simulink model "s_b2a4x1kf"  (R2018b)
settings: Solver=VariableStepDiscrete  StartTime=0.0  StopTime=100  RelTol=1e-3
undefined symbols (not defined in the file): fft_stages, n_bits_ants, n_bits_xengs
libraries: xbsIndex_r4 x20671, casper_library_misc x69, casper_library_scopes x15, casper_library_delays x8, xbsReplacements_r4 x6, xps_library x4
(part 108 of 212)

== system s_b2a4x1kf/sys0/bf/fbf/duplicate ==
  synci : Inport
  eni : Inport  Port=2
  di : Inport  Port=3
  badi : Inport  Port=4
  timei : Inport  Port=5
  misci : Inport  Port=6
  sim_ld : Inport  Port=7
  sim_type : Inport  Port=8
  Convert1 : xbsIndex_r4/Convert  gui_display_data_type=Fixed-point  arith_type=Unsigned  n_bits=n_bits_in*2  bin_pt=0  float_type=Single  exp_bits=8  fraction_bits=24  quantization=Truncate  overflow=Wrap  en=off  latency=0  pipeline=off  dbl_ovrd=off  block_type=convert
      settings: block_version=11.4
  Counter : xbsIndex_r4/Counter  cnt_type=Free Running  cnt_to=inf  operation=Up  start_count=0  cnt_by_val=1  arith_type="Signed  (2's comp)"  n_bits=stack_bits+ant_bits+freq_bits  bin_pt=0  load_pin=off  rst=on  en=on  explicit_period=on  period=1  use_behavioral_HDL=off  implementation=Fabric  dbl_ovrd=off  block_type=counter
      settings: block_version=11.4
  Delay{,1..3,5} (5 alike) : xbsIndex_r4/Delay  rst=off  infoeditControl=Selection of Reset will increase slice count due to use of real FFs and instead of SRLs  en=off  latency=1  reg_retiming=off  dbl_ovrd=off  block_type=delay
      Delay settings: infoedit=Hardware notes: A delay line is a chain, each link of which is an SRL16 or SRL32 followed by a flip-flop.  block_version=11.4
      Delay1 settings: block_version=11.4
      Delay2 settings: block_version=11.4
      Delay3 settings: block_version=11.4
      Delay5 settings: block_version=11.4
  Mux : xbsIndex_r4/Mux  inputs=2  en=off  latency=1  precision=Full  arith_type=Unsigned  n_bits=16  bin_pt=14  quantization=Truncate  overflow=Wrap  dbl_ovrd=off  block_type=mux
      settings: block_version=11.4
  Register1 : xbsIndex_r4/Register  init=0  rst=off  en=on  dbl_ovrd=off  block_type=register
      settings: block_version=11.4
  Slice : xbsIndex_r4/Slice  nbits=freq_bits  boolean_output=off  mode=Upper Bit Location + Width  bit1=0  base1=MSB of Input  bit0=0  base0=LSB of Input  dbl_ovrd=off  block_type=slice
  beam_replicate : Subsystem  Tag=cmac_delinked  mask(bus_replicate){replication=2^beam_bits, csp_latency=0, misc=off, implementation=core}
      mask prompts: replication "replication factor"; csp_latency "latency"; misc "misc support"; implementation "delay implementation"
      mask help: Output bus formed by replicating input bus a number of times
      mask init:
      | bus_replicate_init(gcb, ...
      |     'replication', replication, ...
      |     'csp_latency', csp_latency, ...
      |     'implementation', implementation, ...
      |     'misc', misc);
      mask TypeOptions implementation: core | behavioral
  pol_replicate : Subsystem  Tag=cmac_delinked  mask(bus_replicate){replication=2^polarisation_bits, csp_latency=0, misc=off, implementation=core}
      mask prompts: replication "replication factor"; csp_latency "latency"; misc "misc support"; implementation "delay implementation"
      mask help: Output bus formed by replicating input bus a number of times
      mask init:
      | bus_replicate_init(gcb, ...
      |     'replication', replication, ...
      |     'csp_latency', csp_latency, ...
      |     'implementation', implementation, ...
      |     'misc', misc);
      mask TypeOptions implementation: core | behavioral
  synco : Outport
  do : Outport  Port=2
  eno : Outport  Port=3
  bado : Outport  Port=4
  timeo : Outport  Port=5
  misco : Outport  Port=6
  wires:
  synci/1 -> Delay/1, Counter/1
  eni/1 -> Counter/2, Delay2/1
  badi/1 -> Delay3/1
  misci/1 -> Delay5/1
  timei/1 -> Delay1/1
  Delay/1 -> synco/1
  Delay3/1 -> bado/1
  Delay5/1 -> misco/1
  Delay1/1 -> timeo/1
  sim_ld/1 -> Register1/2
  sim_type/1 -> Register1/1
  beam_replicate/1(out) -> do/1
  Mux/1 -> beam_replicate/1(in)
  Register1/1 -> Mux/1
  di/1 -> Mux/2
  Counter/1 -> Slice/1
  pol_replicate/1(out) -> Mux/3
  Slice/1 -> Convert1/1
  Convert1/1 -> pol_replicate/1(in)
  Delay2/1 -> eno/1

== system s_b2a4x1kf/sys0/bf/fbf/pipeline1 ==
  d : Inport
  Register0 : xbsIndex_r4/Register  init=0  rst=off  en=off  dbl_ovrd=off  block_type=register
      settings: block_version=11.4
  Register1 : xbsIndex_r4/Register  init=0  rst=off  en=off  dbl_ovrd=off  block_type=register
      settings: block_version=11.4
  q : Outport
  wires:
  Register0/1 -> Register1/1
  d/1 -> Register0/1
  Register1/1 -> q/1

== system s_b2a4x1kf/sys0/bf/fbf/pipeline10 ==
  d : Inport
  Register0 : xbsIndex_r4/Register  init=0  rst=off  en=off  dbl_ovrd=off  block_type=register
      settings: block_version=11.4
  Register1 : xbsIndex_r4/Register  init=0  rst=off  en=off  dbl_ovrd=off  block_type=register
      settings: block_version=11.4
  q : Outport
  wires:
  Register0/1 -> Register1/1
  d/1 -> Register0/1
  Register1/1 -> q/1

== system s_b2a4x1kf/sys0/bf/fbf/pipeline11 ==
  d : Inport
  Register0 : xbsIndex_r4/Register  init=0  rst=off  en=off  dbl_ovrd=off  block_type=register
      settings: block_version=11.4
  Register1 : xbsIndex_r4/Register  init=0  rst=off  en=off  dbl_ovrd=off  block_type=register
      settings: block_version=11.4
  q : Outport
  wires:
  Register0/1 -> Register1/1
  d/1 -> Register0/1
  Register1/1 -> q/1

== system s_b2a4x1kf/sys0/bf/fbf/pipeline12 ==
  d : Inport
  Register0 : xbsIndex_r4/Register  init=0  rst=off  en=off  dbl_ovrd=off  block_type=register
      settings: block_version=11.4
  Register1 : xbsIndex_r4/Register  init=0  rst=off  en=off  dbl_ovrd=off  block_type=register
      settings: block_version=11.4
  q : Outport
  wires:
  Register0/1 -> Register1/1
  d/1 -> Register0/1
  Register1/1 -> q/1

== system s_b2a4x1kf/sys0/bf/fbf/pipeline13 ==
  d : Inport
  Register0 : xbsIndex_r4/Register  init=0  rst=off  en=off  dbl_ovrd=off  block_type=register
      settings: block_version=11.4
  Register1 : xbsIndex_r4/Register  init=0  rst=off  en=off  dbl_ovrd=off  block_type=register
      settings: block_version=11.4
  q : Outport
  wires:
  Register0/1 -> Register1/1
  d/1 -> Register0/1
  Register1/1 -> q/1

== system s_b2a4x1kf/sys0/bf/fbf/pipeline14 ==
  d : Inport
  Register0 : xbsIndex_r4/Register  init=0  rst=off  en=off  dbl_ovrd=off  block_type=register
      settings: block_version=11.4
  Register1 : xbsIndex_r4/Register  init=0  rst=off  en=off  dbl_ovrd=off  block_type=register
      settings: block_version=11.4
  q : Outport
  wires:
  Register0/1 -> Register1/1
  d/1 -> Register0/1
  Register1/1 -> q/1

== system s_b2a4x1kf/sys0/bf/fbf/pipeline15 ==
  d : Inport
  Register0 : xbsIndex_r4/Register  init=0  rst=off  en=off  dbl_ovrd=off  block_type=register
      settings: block_version=11.4
  Register1 : xbsIndex_r4/Register  init=0  rst=off  en=off  dbl_ovrd=off  block_type=register
      settings: block_version=11.4
  q : Outport
  wires:
  Register0/1 -> Register1/1
  d/1 -> Register0/1
  Register1/1 -> q/1

== system s_b2a4x1kf/sys0/bf/fbf/pipeline16 ==
  d : Inport
  Register0 : xbsIndex_r4/Register  init=0  rst=off  en=off  dbl_ovrd=off  block_type=register
      settings: block_version=11.4
  Register1 : xbsIndex_r4/Register  init=0  rst=off  en=off  dbl_ovrd=off  block_type=register
      settings: block_version=11.4
  q : Outport
  wires:
  Register0/1 -> Register1/1
  d/1 -> Register0/1
  Register1/1 -> q/1

== system s_b2a4x1kf/sys0/bf/fbf/pipeline2 ==
  d : Inport
  Register0 : xbsIndex_r4/Register  init=0  rst=off  en=off  dbl_ovrd=off  block_type=register
      settings: block_version=11.4
  Register1 : xbsIndex_r4/Register  init=0  rst=off  en=off  dbl_ovrd=off  block_type=register
      settings: block_version=11.4
  q : Outport
  wires:
  Register0/1 -> Register1/1
  d/1 -> Register0/1
  Register1/1 -> q/1

== system s_b2a4x1kf/sys0/bf/fbf/pipeline3 ==
  d : Inport
  Register0 : xbsIndex_r4/Register  init=0  rst=off  en=off  dbl_ovrd=off  block_type=register
      settings: block_version=11.4
  Register1 : xbsIndex_r4/Register  init=0  rst=off  en=off  dbl_ovrd=off  block_type=register
      settings: block_version=11.4
  q : Outport
  wires:
  Register0/1 -> Register1/1
  d/1 -> Register0/1
  Register1/1 -> q/1

== system s_b2a4x1kf/sys0/bf/fbf/pipeline8 ==
  d : Inport
  Register0 : xbsIndex_r4/Register  init=0  rst=off  en=off  dbl_ovrd=off  block_type=register
      settings: block_version=11.4
  Register1 : xbsIndex_r4/Register  init=0  rst=off  en=off  dbl_ovrd=off  block_type=register
      settings: block_version=11.4
  q : Outport
  wires:
  Register0/1 -> Register1/1
  d/1 -> Register0/1
  Register1/1 -> q/1

== system s_b2a4x1kf/sys0/bf/fbf/pipeline9 ==
  d : Inport
  Register0 : xbsIndex_r4/Register  init=0  rst=off  en=off  dbl_ovrd=off  block_type=register
      settings: block_version=11.4
  Register1 : xbsIndex_r4/Register  init=0  rst=off  en=off  dbl_ovrd=off  block_type=register
      settings: block_version=11.4
  q : Outport
  wires:
  Register0/1 -> Register1/1
  d/1 -> Register0/1
  Register1/1 -> q/1

== system s_b2a4x1kf/sys0/bf/fbf/requantise ==
  synci : Inport
  din : Inport  Port=2
  den : Inport  Port=3
  misci : Inport  Port=4
  vali : Inport  Port=5
  Concat : xbsIndex_r4/Concat  num_inputs=3  dbl_ovrd=off  block_type=concat
  Slice : xbsIndex_r4/Slice  nbits=1  boolean_output=on  mode=Upper Bit Location + Width  bit1=-1  base1=MSB of Input  bit0=0  base0=LSB of Input  dbl_ovrd=off  block_type=slice
  Slice1 : xbsIndex_r4/Slice  nbits=1  boolean_output=off  mode=Two Bit Locations  bit1=-2  base1=MSB of Input  bit0=0  base0=LSB of Input  dbl_ovrd=off  block_type=slice
  Slice2 : xbsIndex_r4/Slice  nbits=1  boolean_output=on  mode=Upper Bit Location + Width  bit1=0  base1=MSB of Input  bit0=0  base0=LSB of Input  dbl_ovrd=off  block_type=slice
  bus_convert : Subsystem  Tag=cmac_delinked  mask(bus_convert){n_bits_in=repmat(n_bits_coeff+n_bits_in+1, 1, 2^stream_bits), bin_pt_in=bin_pt_coeff+bin_pt_in, cmplx=on, n_bits_out=n_bits_out, bin_pt_out=bin_pt_out, quantization=quantization, overflow=overflow, csp_latency=conv_latency, of=off, misc=on}
      mask prompts: n_bits_in "input bit widths"; bin_pt_in "input binary points"; cmplx "input complex"; n_bits_out "output bit widths"; bin_pt_out "output binary points"; quantization "quantization strategy (Truncate=0, Round  (unbiased: +/- Inf)=1, Round (unbiased: Even Values)=2)"; overflow "overflow strategy (Wrap=0, Saturate=1, Flag as error=2)"; csp_latency "latency"; of "overflow indication"; misc "misc support"
      mask help: Convert components of busses
      mask init: same as s_b2a4x1kf/sys0/31->32
  bus_mult : Subsystem  mask(bus_mult){n_bits_a=repmat(n_bits_in, 1, 2^stream_bits), bin_pt_a=bin_pt_in, type_a=type_in, cmplx_a=on, n_bits_b=repmat(n_bits_coeff, 1, 2^stream_bits), bin_pt_b=bin_pt_coeff, type_b=type_coeff, cmplx_b=off, n_bits_out=n_bits_coeff+n_bits_in+1, bin_pt_out=bin_pt_coeff+bin_pt_in, type_out=type_out, quantization=0, overflow=0, mult_latency=mult_latency, add_latency=2, conv_latency=0, max_fanout=2, fan_latency=1, multiplier_implementation=embedded multiplier core, misc=on}
      mask prompts: n_bits_a "a input bit widths"; bin_pt_a "a input binary points"; type_a "a input type (Unsigned=0, Signed=1)"; cmplx_a "a input complex"; n_bits_b "b input bit widths"; bin_pt_b "b input binary points"; type_b "b input type (Unsigned=0, Signed=1)"; cmplx_b "b input complex"; n_bits_out "output bit widths"; bin_pt_out "output binary points"; type_out "output type (Unsigned=0, Signed=1)"; quantization "quantization strategy (Truncate=0, Round  (unbiased: +/- Inf)=1)"; overflow "overflow strategy (Wrap=0, Saturate=1, Flag as error=2)"; mult_latency "multiplier latency"; add_latency "adder latency"; conv_latency "convert latency"; max_fanout "limit fanout to ?"; fan_latency "fanout register latency"; multiplier_implementation "multiplier implementation"; misc "misc support"
      mask help: Multiply components of two busses
      mask init: same as s_b2a4x1kf/sys0/bf/fbf/apply_beam_weights/bus_mult
      mask TypeOptions multiplier_implementation: behavioral HDL | standard core | embedded multiplier core
  synco : Outport
  dout : Outport  Port=2
  eno : Outport  Port=3
  misco : Outport  Port=4
  wires:
  bus_convert/1(dout) -> dout/1
  vali/1 -> bus_mult/2(b)
  Slice2/1 -> synco/1
  misci/1 -> Concat/3
  bus_convert/2(misco) -> Slice1/1, Slice2/1, Slice/1
  Slice1/1 -> misco/1
  Slice/1 -> eno/1
  synci/1 -> Concat/1
  den/1 -> Concat/2
  din/1 -> bus_mult/1(a)
  bus_mult/1(a*b) -> bus_convert/1(din)
  Concat/1 -> bus_mult/3(misci)
  bus_mult/2(misco) -> bus_convert/2(misci)

== system s_b2a4x1kf/sys0/bf/fbf/sync_gen ==
  en : Inport
  di : Inport  Port=2
  badi : Inport  Port=3
  timei : Inport  Port=4
  misci : Inport  Port=5
  Delay{,1..10} (11 alike) : xbsIndex_r4/Delay  rst=off  infoeditControl=Selection of Reset will increase slice count due to use of real FFs and instead of SRLs  en=off  latency=1  reg_retiming=on  dbl_ovrd=off  block_type=delay
  different_time : xbsIndex_r4/Relational  mode=a!=b  op_type=Bool  en=off  latency=0  dbl_ovrd=off  block_type=relational
  pre_time : xbsIndex_r4/Register  init=0  rst=off  en=off  dbl_ovrd=off  block_type=register
  synco : Outport
  do : Outport  Port=2
  dvalid : Outport  Port=3
  bado : Outport  Port=4
  timeo : Outport  Port=5
  misco : Outport  Port=6
  wires:
  Delay9/1 -> misco/1
  Delay7/1 -> bado/1
  Delay8/1 -> do/1
  Delay3/1 -> Delay9/1
  Delay2/1 -> Delay7/1
  Delay1/1 -> Delay8/1
  Delay4/1 -> dvalid/1
  Delay6/1 -> timeo/1
  Delay5/1 -> Delay6/1
  different_time/1 -> Delay10/1
  Delay/1 -> Delay4/1
  badi/1 -> Delay2/1
  misci/1 -> Delay3/1
  di/1 -> Delay1/1
  en/1 -> Delay/1
  pre_time/1 -> different_time/2
  timei/1 -> Delay5/1, pre_time/1, different_time/1
  Delay10/1 -> synco/1

== system s_b2a4x1kf/sys0/bf_pack_out0/Subsystem3/edge_detect ==
  in : Inport
  Delay : xbsIndex_r4/Delay  rst=off  infoeditControl=Selection of Reset will increase slice count due to use of real FFs and instead of SRLs  en=off  latency=1  reg_retiming=off  dbl_ovrd=off  block_type=delay
      settings: xl_area=[0, 0, 0, 0, 0, 0, 0]
  Inverter : xbsIndex_r4/Inverter  en=off  latency=0  dbl_ovrd=off  block_type=inv
      settings: xl_area=[0, 0, 0, 0, 0, 0, 0]
  edge_op : xbsIndex_r4/Logical  logical_function=NOR  inputs=2  en=off  latency=0  precision=Full  arith_type=Unsigned  n_bits=8  bin_pt=2  align_bp=on  dbl_ovrd=off  block_type=logical
      settings: xl_area=[0, 0, 0, 0, 0, 0, 0]
  out : Outport
  wires:
  Inverter/1 -> edge_op/1
  edge_op/1 -> out/1
  in/1 -> Inverter/1, Delay/1
  Delay/1 -> edge_op/2

== system s_b2a4x1kf/sys0/bf_pack_out0/Subsystem3/edge_detect1 ==
  in : Inport
  Delay : xbsIndex_r4/Delay  rst=off  infoeditControl=Selection of Reset will increase slice count due to use of real FFs and instead of SRLs  en=off  latency=1  reg_retiming=off  dbl_ovrd=off  block_type=delay
      settings: xl_area=[0, 0, 0, 0, 0, 0, 0]
  Inverter : xbsIndex_r4/Inverter  en=off  latency=0  dbl_ovrd=off  block_type=inv
      settings: xl_area=[0, 0, 0, 0, 0, 0, 0]
  edge_op : xbsIndex_r4/Logical  logical_function=NOR  inputs=2  en=off  latency=0  precision=Full  arith_type=Unsigned  n_bits=8  bin_pt=2  align_bp=on  dbl_ovrd=off  block_type=logical
      settings: xl_area=[0, 0, 0, 0, 0, 0, 0]
  out : Outport
  wires:
  Inverter/1 -> edge_op/1
  edge_op/1 -> out/1
  in/1 -> Inverter/1, Delay/1
  Delay/1 -> edge_op/2

== system s_b2a4x1kf/sys0/bf_pack_out0/Subsystem3/pipeline1 ==
  d : Inport
  Register0 : xbsIndex_r4/Register  init=0  rst=off  en=off  dbl_ovrd=off  block_type=register
      settings: block_version=11.4
  Register1 : xbsIndex_r4/Register  init=0  rst=off  en=off  dbl_ovrd=off  block_type=register
      settings: block_version=11.4
  q : Outport
  wires:
  Register0/1 -> Register1/1
  d/1 -> Register0/1
  Register1/1 -> q/1

== system s_b2a4x1kf/sys0/bf_pack_out0/Subsystem3/pipeline2 ==
  d : Inport
  Register0 : xbsIndex_r4/Register  init=0  rst=off  en=off  dbl_ovrd=off  block_type=register
      settings: block_version=11.4
  Register1 : xbsIndex_r4/Register  init=0  rst=off  en=off  dbl_ovrd=off  block_type=register
      settings: block_version=11.4
  q : Outport
  wires:
  Register0/1 -> Register1/1
  d/1 -> Register0/1
  Register1/1 -> q/1

== system s_b2a4x1kf/sys0/bf_pack_out0/Subsystem3/pipeline53 ==
  d : Inport
  Register0 : xbsIndex_r4/Register  init=0  rst=off  en=off  dbl_ovrd=off  block_type=register
      settings: block_version=11.4
  Register1 : xbsIndex_r4/Register  init=0  rst=off  en=off  dbl_ovrd=off  block_type=register
      settings: block_version=11.4
  q : Outport
  wires:
  Register0/1 -> Register1/1
  d/1 -> Register0/1
  Register1/1 -> q/1

== system s_b2a4x1kf/sys0/bf_pack_out0/Subsystem3/pipeline54 ==
  d : Inport
  Register0 : xbsIndex_r4/Register  init=0  rst=off  en=off  dbl_ovrd=off  block_type=register
      settings: block_version=11.4
  Register1 : xbsIndex_r4/Register  init=0  rst=off  en=off  dbl_ovrd=off  block_type=register
      settings: block_version=11.4
  q : Outport
  wires:
  Register0/1 -> Register1/1
  d/1 -> Register0/1
  Register1/1 -> q/1

== system s_b2a4x1kf/sys0/bf_pack_out0/Subsystem3/pipeline55 ==
  d : Inport
  Register0 : xbsIndex_r4/Register  init=0  rst=off  en=off  dbl_ovrd=off  block_type=register
      settings: block_version=11.4
  Register1 : xbsIndex_r4/Register  init=0  rst=off  en=off  dbl_ovrd=off  block_type=register
      settings: block_version=11.4
  q : Outport
  wires:
  Register0/1 -> Register1/1
  d/1 -> Register0/1
  Register1/1 -> q/1

== system s_b2a4x1kf/sys0/bf_pack_out0/Subsystem3/pipeline7 ==
  d : Inport
  Register0 : xbsIndex_r4/Register  init=0  rst=off  en=off  dbl_ovrd=off  block_type=register
      settings: block_version=11.4
  Register1 : xbsIndex_r4/Register  init=0  rst=off  en=off  dbl_ovrd=off  block_type=register
      settings: block_version=11.4
  q : Outport
  wires:
  Register0/1 -> Register1/1
  d/1 -> Register0/1
  Register1/1 -> q/1

== system s_b2a4x1kf/sys0/bf_pack_out0/data_fifo/bus_replicate ==
  in : Inport
  bussify : Subsystem  mask(bus_create){inputNum=16}
      mask prompts: inputNum "Number of inputs:"
      mask init:
      | bus_create_init(gcb,...
      |     'inputNum', inputNum);
  out : Outport
  wires:
  in/1 -> bussify/1(in1), bussify/2(in2), bussify/3(in3), bussify/4(in4), bussify/5(in5), bussify/6(in6), bussify/7(in7), bussify/8(in8), bussify/9(in9), bussify/10(in10), bussify/11(in11), bussify/12(in12), bussify/13(in13), bussify/14(in14), bussify/15(in15), bussify/16(in16)
  bussify/1(bus_out) -> out/1

== system s_b2a4x1kf/sys0/bf_pack_out0/data_fifo/edge_detect ==
  in : Inport
  Delay : xbsIndex_r4/Delay  rst=off  infoeditControl=Selection of Reset will increase slice count due to use of real FFs and instead of SRLs  en=off  latency=1  reg_retiming=on  dbl_ovrd=off  block_type=delay
      settings: xl_area=[0, 0, 0, 0, 0, 0, 0]
  Inverter : xbsIndex_r4/Inverter  en=off  latency=0  dbl_ovrd=off  block_type=inv
      settings: xl_area=[0, 0, 0, 0, 0, 0, 0]
  edge_op : xbsIndex_r4/Logical  logical_function=AND  inputs=2  en=off  latency=0  precision=Full  arith_type=Unsigned  n_bits=8  bin_pt=2  align_bp=on  dbl_ovrd=off  block_type=logical
      settings: xl_area=[0, 0, 0, 0, 0, 0, 0]
  out : Outport
  wires:
  Inverter/1 -> edge_op/1
  edge_op/1 -> out/1
  in/1 -> Inverter/1, Delay/1
  Delay/1 -> edge_op/2

== system s_b2a4x1kf/sys0/bf_pack_out0/data_fifo/edge_detect1 ==
  in : Inport
  Delay : xbsIndex_r4/Delay  rst=off  infoeditControl=Selection of Reset will increase slice count due to use of real FFs and instead of SRLs  en=off  latency=1  reg_retiming=on  dbl_ovrd=off  block_type=delay
      settings: xl_area=[0, 0, 0, 0, 0, 0, 0]
  Inverter : xbsIndex_r4/Inverter  en=off  latency=0  dbl_ovrd=off  block_type=inv
      settings: xl_area=[0, 0, 0, 0, 0, 0, 0]
  edge_op : xbsIndex_r4/Logical  logical_function=AND  inputs=2  en=off  latency=0  precision=Full  arith_type=Unsigned  n_bits=8  bin_pt=2  align_bp=on  dbl_ovrd=off  block_type=logical
      settings: xl_area=[0, 0, 0, 0, 0, 0, 0]
  out : Outport
  wires:
  Delay/1 -> edge_op/2
  in/1 -> Delay/1, Inverter/1
  edge_op/1 -> out/1
  Inverter/1 -> edge_op/1

== system s_b2a4x1kf/sys0/bf_pack_out0/data_fifo/munge ==
  din : Inport
  join : Subsystem  mask(bus_create){inputNum=16}
      mask prompts: inputNum "Number of inputs:"
      mask init:
      | bus_create_init(gcb,...
      |     'inputNum', inputNum);
  reinterpret : xbsIndex_r4/Reinterpret  force_arith_type=on  arith_type=Unsigned  force_bin_pt=on  bin_pt=0  block_type=reinterpret
      settings: infoedit="Changes signal type without altering the binary representation.   You can changed the signal between signed and unsigned, and relocate the binary point.<br><br>Hardware notes: In hardware this block costs nothing.<br><br>Example:  Suppose the input is 6 bits wide, signed, with 2 fractional bits, and the output is forced to unsigned with 0 fractional bits.  Then an input of -2.0 (1110.00 in binary 2's complement) becomes an output of 56 (111000 in binary)."
  reinterpret_out : xbsIndex_r4/Reinterpret  force_arith_type=on  arith_type=Unsigned  force_bin_pt=on  bin_pt=0  block_type=reinterpret
  split : Subsystem  mask(bus_expand){mode=divisions of arbitrary size, outputNum=1, outputWidth=[16 16 16 16 16 16 16 16 16 16 16 16 16 16 16 16], outputBinaryPt=[0 0 0 0 0 0 0 0 0 0 0 0 0 0 0 0], outputArithmeticType=[0 0 0 0 0 0 0 0 0 0 0 0 0 0 0 0], show_format=off, outputToWorkspace=off, variablePrefix=out, outputToModelAsWell=on}
      mask prompts: outputNum "Number of outputs:"; outputWidth "Output width [msb ... lsb]:"; outputBinaryPt "Output binary point position [msb ... lsb]:"; outputArithmeticType "Output arithmetic type (ufix=0, fix=1, bool=2) [msb ... lsb]:"; show_format "Print format string?"; outputToWorkspace "Output to workspace?"; variablePrefix "Variable name prefix:"; outputToModelAsWell "Output to model as well?"
      mask help:
      | Expands a 'bus' made using a bus_create or Xilinx
      | concat block.
      | The input will be divided into the specified number
      | of outputs with the specified arithmetic types.
      | Divisions are made from most significant bit.
      mask init: same as s_b2a4x1kf/bus_expand
      settings: AttributesFormatString=16 outputs
      mask TypeOptions mode: divisions of equal size | divisions of arbitrary size
      mask Callback mode: bus_expand_callback();
      mask Callback outputWidth: bus_expand_callback();
      mask Callback outputToWorkspace: bus_expand_callback();
  dout : Outport
  wires:
  reinterpret_out/1 -> dout/1
  din/1 -> reinterpret/1
  reinterpret/1 -> split/1(bus_in)
  join/1(bus_out) -> reinterpret_out/1
  split/16(lsb_out1) -> join/1(in1)
  split/15(out2) -> join/2(in2)
  split/14(out3) -> join/3(in3)
  split/13(out4) -> join/4(in4)
  split/12(out5) -> join/5(in5)
  split/11(out6) -> join/6(in6)
  split/10(out7) -> join/7(in7)
  split/9(out8) -> join/8(in8)
  split/8(out9) -> join/9(in9)
  split/7(out10) -> join/10(in10)
  split/6(out11) -> join/11(in11)
  split/5(out12) -> join/12(in12)
  split/4(out13) -> join/13(in13)
  split/3(out14) -> join/14(in14)
  split/2(out15) -> join/15(in15)
  split/1(msb_out16) -> join/16(in16)

== system s_b2a4x1kf/sys0/bf_pack_out0/pack/edge_detect1 ==
  in : Inport
  Delay : xbsIndex_r4/Delay  rst=off  infoeditControl=Selection of Reset will increase slice count due to use of real FFs and instead of SRLs  en=off  latency=1  reg_retiming=on  dbl_ovrd=off  block_type=delay
      settings: xl_area=[0, 0, 0, 0, 0, 0, 0]
  Inverter : xbsIndex_r4/Inverter  en=off  latency=0  dbl_ovrd=off  block_type=inv
      settings: xl_area=[0, 0, 0, 0, 0, 0, 0]
  edge_op : xbsIndex_r4/Logical  logical_function=AND  inputs=2  en=off  latency=0  precision=Full  arith_type=Unsigned  n_bits=8  bin_pt=2  align_bp=on  dbl_ovrd=off  block_type=logical
      settings: xl_area=[0, 0, 0, 0, 0, 0, 0]
  out : Outport
  wires:
  Delay/1 -> edge_op/2
  in/1 -> Delay/1, Inverter/1
  edge_op/1 -> out/1
  Inverter/1 -> edge_op/1

== system s_b2a4x1kf/sys0/bf_pack_out0/pack/edge_detect3 ==
  in : Inport
  Delay : xbsIndex_r4/Delay  rst=off  infoeditControl=Selection of Reset will increase slice count due to use of real FFs and instead of SRLs  en=off  latency=1  reg_retiming=on  dbl_ovrd=off  block_type=delay
      settings: xl_area=[0, 0, 0, 0, 0, 0, 0]
  Inverter : xbsIndex_r4/Inverter  en=off  latency=0  dbl_ovrd=off  block_type=inv
      settings: xl_area=[0, 0, 0, 0, 0, 0, 0]
  edge_op : xbsIndex_r4/Logical  logical_function=NOR  inputs=2  en=off  latency=0  precision=Full  arith_type=Unsigned  n_bits=8  bin_pt=2  align_bp=on  dbl_ovrd=off  block_type=logical
      settings: xl_area=[0, 0, 0, 0, 0, 0, 0]
  out : Outport
  wires:
  Delay/1 -> edge_op/2
  in/1 -> Delay/1, Inverter/1
  edge_op/1 -> out/1
  Inverter/1 -> edge_op/1

== system s_b2a4x1kf/sys0/bf_pack_out1/Subsystem3/edge_detect ==
  in : Inport
  Delay : xbsIndex_r4/Delay  rst=off  infoeditControl=Selection of Reset will increase slice count due to use of real FFs and instead of SRLs  en=off  latency=1  reg_retiming=off  dbl_ovrd=off  block_type=delay
      settings: xl_area=[0, 0, 0, 0, 0, 0, 0]
  Inverter : xbsIndex_r4/Inverter  en=off  latency=0  dbl_ovrd=off  block_type=inv
      settings: xl_area=[0, 0, 0, 0, 0, 0, 0]
  edge_op : xbsIndex_r4/Logical  logical_function=NOR  inputs=2  en=off  latency=0  precision=Full  arith_type=Unsigned  n_bits=8  bin_pt=2  align_bp=on  dbl_ovrd=off  block_type=logical
      settings: xl_area=[0, 0, 0, 0, 0, 0, 0]
  out : Outport
  wires:
  Inverter/1 -> edge_op/1
  edge_op/1 -> out/1
  in/1 -> Inverter/1, Delay/1
  Delay/1 -> edge_op/2

== system s_b2a4x1kf/sys0/bf_pack_out1/Subsystem3/edge_detect1 ==
  in : Inport
  Delay : xbsIndex_r4/Delay  rst=off  infoeditControl=Selection of Reset will increase slice count due to use of real FFs and instead of SRLs  en=off  latency=1  reg_retiming=off  dbl_ovrd=off  block_type=delay
      settings: xl_area=[0, 0, 0, 0, 0, 0, 0]
  Inverter : xbsIndex_r4/Inverter  en=off  latency=0  dbl_ovrd=off  block_type=inv
      settings: xl_area=[0, 0, 0, 0, 0, 0, 0]
  edge_op : xbsIndex_r4/Logical  logical_function=NOR  inputs=2  en=off  latency=0  precision=Full  arith_type=Unsigned  n_bits=8  bin_pt=2  align_bp=on  dbl_ovrd=off  block_type=logical
      settings: xl_area=[0, 0, 0, 0, 0, 0, 0]
  out : Outport
  wires:
  Inverter/1 -> edge_op/1
  edge_op/1 -> out/1
  in/1 -> Inverter/1, Delay/1
  Delay/1 -> edge_op/2

== system s_b2a4x1kf/sys0/bf_pack_out1/Subsystem3/pipeline1 ==
  d : Inport
  Register0 : xbsIndex_r4/Register  init=0  rst=off  en=off  dbl_ovrd=off  block_type=register
      settings: block_version=11.4
  Register1 : xbsIndex_r4/Register  init=0  rst=off  en=off  dbl_ovrd=off  block_type=register
      settings: block_version=11.4
  q : Outport
  wires:
  Register0/1 -> Register1/1
  d/1 -> Register0/1
  Register1/1 -> q/1

== system s_b2a4x1kf/sys0/bf_pack_out1/Subsystem3/pipeline2 ==
  d : Inport
  Register0 : xbsIndex_r4/Register  init=0  rst=off  en=off  dbl_ovrd=off  block_type=register
      settings: block_version=11.4
  Register1 : xbsIndex_r4/Register  init=0  rst=off  en=off  dbl_ovrd=off  block_type=register
      settings: block_version=11.4
  q : Outport
  wires:
  Register0/1 -> Register1/1
  d/1 -> Register0/1
  Register1/1 -> q/1

== system s_b2a4x1kf/sys0/bf_pack_out1/Subsystem3/pipeline53 ==
  d : Inport
  Register0 : xbsIndex_r4/Register  init=0  rst=off  en=off  dbl_ovrd=off  block_type=register
      settings: block_version=11.4
  Register1 : xbsIndex_r4/Register  init=0  rst=off  en=off  dbl_ovrd=off  block_type=register
      settings: block_version=11.4
  q : Outport
  wires:
  Register0/1 -> Register1/1
  d/1 -> Register0/1
  Register1/1 -> q/1

== system s_b2a4x1kf/sys0/bf_pack_out1/Subsystem3/pipeline54 ==
  d : Inport
  Register0 : xbsIndex_r4/Register  init=0  rst=off  en=off  dbl_ovrd=off  block_type=register
      settings: block_version=11.4
  Register1 : xbsIndex_r4/Register  init=0  rst=off  en=off  dbl_ovrd=off  block_type=register
      settings: block_version=11.4
  q : Outport
  wires:
  Register0/1 -> Register1/1
  d/1 -> Register0/1
  Register1/1 -> q/1

== system s_b2a4x1kf/sys0/bf_pack_out1/Subsystem3/pipeline55 ==
  d : Inport
  Register0 : xbsIndex_r4/Register  init=0  rst=off  en=off  dbl_ovrd=off  block_type=register
      settings: block_version=11.4
  Register1 : xbsIndex_r4/Register  init=0  rst=off  en=off  dbl_ovrd=off  block_type=register
      settings: block_version=11.4
  q : Outport
  wires:
  Register0/1 -> Register1/1
  d/1 -> Register0/1
  Register1/1 -> q/1

== system s_b2a4x1kf/sys0/bf_pack_out1/Subsystem3/pipeline7 ==
  d : Inport
  Register0 : xbsIndex_r4/Register  init=0  rst=off  en=off  dbl_ovrd=off  block_type=register
      settings: block_version=11.4
  Register1 : xbsIndex_r4/Register  init=0  rst=off  en=off  dbl_ovrd=off  block_type=register
      settings: block_version=11.4
  q : Outport
  wires:
  Register0/1 -> Register1/1
  d/1 -> Register0/1
  Register1/1 -> q/1

== system s_b2a4x1kf/sys0/bf_pack_out1/data_fifo/bus_replicate ==
  in : Inport
  bussify : Subsystem  mask(bus_create){inputNum=16}
      mask prompts: inputNum "Number of inputs:"
      mask init:
      | bus_create_init(gcb,...
      |     'inputNum', inputNum);
  out : Outport
  wires:
  in/1 -> bussify/1(in1), bussify/2(in2), bussify/3(in3), bussify/4(in4), bussify/5(in5), bussify/6(in6), bussify/7(in7), bussify/8(in8), bussify/9(in9), bussify/10(in10), bussify/11(in11), bussify/12(in12), bussify/13(in13), bussify/14(in14), bussify/15(in15), bussify/16(in16)
  bussify/1(bus_out) -> out/1

== system s_b2a4x1kf/sys0/bf_pack_out1/data_fifo/edge_detect ==
  in : Inport
  Delay : xbsIndex_r4/Delay  rst=off  infoeditControl=Selection of Reset will increase slice count due to use of real FFs and instead of SRLs  en=off  latency=1  reg_retiming=on  dbl_ovrd=off  block_type=delay
      settings: xl_area=[0, 0, 0, 0, 0, 0, 0]
  Inverter : xbsIndex_r4/Inverter  en=off  latency=0  dbl_ovrd=off  block_type=inv
      settings: xl_area=[0, 0, 0, 0, 0, 0, 0]
  edge_op : xbsIndex_r4/Logical  logical_function=AND  inputs=2  en=off  latency=0  precision=Full  arith_type=Unsigned  n_bits=8  bin_pt=2  align_bp=on  dbl_ovrd=off  block_type=logical
      settings: xl_area=[0, 0, 0, 0, 0, 0, 0]
  out : Outport
  wires:
  Delay/1 -> edge_op/2
  in/1 -> Delay/1, Inverter/1
  edge_op/1 -> out/1
  Inverter/1 -> edge_op/1

== system s_b2a4x1kf/sys0/bf_pack_out1/data_fifo/edge_detect1 ==
  in : Inport
  Delay : xbsIndex_r4/Delay  rst=off  infoeditControl=Selection of Reset will increase slice count due to use of real FFs and instead of SRLs  en=off  latency=1  reg_retiming=on  dbl_ovrd=off  block_type=delay
      settings: xl_area=[0, 0, 0, 0, 0, 0, 0]
  Inverter : xbsIndex_r4/Inverter  en=off  latency=0  dbl_ovrd=off  block_type=inv
      settings: xl_area=[0, 0, 0, 0, 0, 0, 0]
  edge_op : xbsIndex_r4/Logical  logical_function=AND  inputs=2  en=off  latency=0  precision=Full  arith_type=Unsigned  n_bits=8  bin_pt=2  align_bp=on  dbl_ovrd=off  block_type=logical
      settings: xl_area=[0, 0, 0, 0, 0, 0, 0]
  out : Outport
  wires:
  Inverter/1 -> edge_op/1
  edge_op/1 -> out/1
  in/1 -> Inverter/1, Delay/1
  Delay/1 -> edge_op/2

== system s_b2a4x1kf/sys0/bf_pack_out1/data_fifo/munge ==
  din : Inport
  join : Subsystem  mask(bus_create){inputNum=16}
      mask prompts: inputNum "Number of inputs:"
      mask init:
      | bus_create_init(gcb,...
      |     'inputNum', inputNum);
  reinterpret : xbsIndex_r4/Reinterpret  force_arith_type=on  arith_type=Unsigned  force_bin_pt=on  bin_pt=0  block_type=reinterpret
      settings: infoedit="Changes signal type without altering the binary representation.   You can changed the signal between signed and unsigned, and relocate the binary point.<br><br>Hardware notes: In hardware this block costs nothing.<br><br>Example:  Suppose the input is 6 bits wide, signed, with 2 fractional bits, and the output is forced to unsigned with 0 fractional bits.  Then an input of -2.0 (1110.00 in binary 2's complement) becomes an output of 56 (111000 in binary)."
  reinterpret_out : xbsIndex_r4/Reinterpret  force_arith_type=on  arith_type=Unsigned  force_bin_pt=on  bin_pt=0  block_type=reinterpret
  split : Subsystem  mask(bus_expand){mode=divisions of arbitrary size, outputNum=1, outputWidth=[16 16 16 16 16 16 16 16 16 16 16 16 16 16 16 16], outputBinaryPt=[0 0 0 0 0 0 0 0 0 0 0 0 0 0 0 0], outputArithmeticType=[0 0 0 0 0 0 0 0 0 0 0 0 0 0 0 0], show_format=off, outputToWorkspace=off, variablePrefix=out, outputToModelAsWell=on}
      mask prompts: outputNum "Number of outputs:"; outputWidth "Output width [msb ... lsb]:"; outputBinaryPt "Output binary point position [msb ... lsb]:"; outputArithmeticType "Output arithmetic type (ufix=0, fix=1, bool=2) [msb ... lsb]:"; show_format "Print format string?"; outputToWorkspace "Output to workspace?"; variablePrefix "Variable name prefix:"; outputToModelAsWell "Output to model as well?"
      mask help:
      | Expands a 'bus' made using a bus_create or Xilinx
      | concat block.
      | The input will be divided into the specified number
      | of outputs with the specified arithmetic types.
      | Divisions are made from most significant bit.
      mask init: same as s_b2a4x1kf/bus_expand
      settings: AttributesFormatString=16 outputs
      mask TypeOptions mode: divisions of equal size | divisions of arbitrary size
      mask Callback mode: bus_expand_callback();
      mask Callback outputWidth: bus_expand_callback();
      mask Callback outputToWorkspace: bus_expand_callback();
  dout : Outport
  wires:
  split/1(msb_out16) -> join/16(in16)
  split/2(out15) -> join/15(in15)
  split/3(out14) -> join/14(in14)
  split/4(out13) -> join/13(in13)
  split/5(out12) -> join/12(in12)
  split/6(out11) -> join/11(in11)
  split/7(out10) -> join/10(in10)
  split/8(out9) -> join/9(in9)
  split/9(out8) -> join/8(in8)
  split/10(out7) -> join/7(in7)
  split/11(out6) -> join/6(in6)
  split/12(out5) -> join/5(in5)
  split/13(out4) -> join/4(in4)
  split/14(out3) -> join/3(in3)
  split/15(out2) -> join/2(in2)
  split/16(lsb_out1) -> join/1(in1)
  join/1(bus_out) -> reinterpret_out/1
  reinterpret/1 -> split/1(bus_in)
  din/1 -> reinterpret/1
  reinterpret_out/1 -> dout/1

== system s_b2a4x1kf/sys0/bf_pack_out1/pack/edge_detect1 ==
  in : Inport
  Delay : xbsIndex_r4/Delay  rst=off  infoeditControl=Selection of Reset will increase slice count due to use of real FFs and instead of SRLs  en=off  latency=1  reg_retiming=on  dbl_ovrd=off  block_type=delay
      settings: xl_area=[0, 0, 0, 0, 0, 0, 0]
  Inverter : xbsIndex_r4/Inverter  en=off  latency=0  dbl_ovrd=off  block_type=inv
      settings: xl_area=[0, 0, 0, 0, 0, 0, 0]
  edge_op : xbsIndex_r4/Logical  logical_function=AND  inputs=2  en=off  latency=0  precision=Full  arith_type=Unsigned  n_bits=8  bin_pt=2  align_bp=on  dbl_ovrd=off  block_type=logical
      settings: xl_area=[0, 0, 0, 0, 0, 0, 0]
  out : Outport
  wires:
  Inverter/1 -> edge_op/1
  edge_op/1 -> out/1
  in/1 -> Inverter/1, Delay/1
  Delay/1 -> edge_op/2

== system s_b2a4x1kf/sys0/bf_pack_out1/pack/edge_detect3 ==
  in : Inport
  Delay : xbsIndex_r4/Delay  rst=off  infoeditControl=Selection of Reset will increase slice count due to use of real FFs and instead of SRLs  en=off  latency=1  reg_retiming=on  dbl_ovrd=off  block_type=delay
      settings: xl_area=[0, 0, 0, 0, 0, 0, 0]
  Inverter : xbsIndex_r4/Inverter  en=off  latency=0  dbl_ovrd=off  block_type=inv
      settings: xl_area=[0, 0, 0, 0, 0, 0, 0]
  edge_op : xbsIndex_r4/Logical  logical_function=NOR  inputs=2  en=off  latency=0  precision=Full  arith_type=Unsigned  n_bits=8  bin_pt=2  align_bp=on  dbl_ovrd=off  block_type=logical
      settings: xl_area=[0, 0, 0, 0, 0, 0, 0]
  out : Outport
  wires:
  Inverter/1 -> edge_op/1
  edge_op/1 -> out/1
  in/1 -> Inverter/1, Delay/1
  Delay/1 -> edge_op/2

== system s_b2a4x1kf/sys0/pkt_reord/bus_replicate/bussify ==
  in1 : Inport
  reinterpret1 : xbsIndex_r4/Reinterpret  force_arith_type=on  arith_type=Unsigned  force_bin_pt=on  bin_pt=0  block_type=reinterpret
      settings: infoedit="Changes signal type without altering the binary representation.   You can changed the signal between signed and unsigned, and relocate the binary point.<br><br>Hardware notes: In hardware this block costs nothing.<br><br>Example:  Suppose the input is 6 bits wide, signed, with 2 fractional bits, and the output is forced to unsigned with 0 fractional bits.  Then an input of -2.0 (1110.00 in binary 2's complement) becomes an output of 56 (111000 in binary)."
  bus_out : Outport
  wires:
  in1/1 -> reinterpret1/1
  reinterpret1/1 -> bus_out/1

== system s_b2a4x1kf/sys0/pkt_reord/input_control/adder_tree ==
  sync : Inport
  din1 : Inport  Port=2
  din2 : Inport  Port=3
  din3 : Inport  Port=4
  addr1 : xbsIndex_r4/AddSub  mode=Addition  use_carryin=off  use_carryout=off  en=off  latency=2  precision=Full  arith_type=Unsigned  n_bits=16  bin_pt=14  quantization=Truncate  overflow=Wrap  use_behavioral_HDL=off  hw_selection=Fabric  pipelined=on  use_rpm=on  dbl_ovrd=off  block_type=addsub
  addr3 : xbsIndex_r4/AddSub  mode=Addition  use_carryin=off  use_carryout=off  en=off  latency=2  precision=Full  arith_type=Unsigned  n_bits=16  bin_pt=14  quantization=Truncate  overflow=Wrap  use_behavioral_HDL=off  hw_selection=Fabric  pipelined=on  use_rpm=on  dbl_ovrd=off  block_type=addsub
  dly2 : xbsIndex_r4/Delay  rst=off  infoeditControl=Selection of Reset will increase slice count due to use of real FFs and instead of SRLs  en=off  latency=2  reg_retiming=on  dbl_ovrd=off  block_type=delay
  sync_delay : xbsIndex_r4/Delay  rst=off  infoeditControl=Selection of Reset will increase slice count due to use of real FFs and instead of SRLs  en=off  latency=4  reg_retiming=on  dbl_ovrd=off  block_type=delay
      settings: block_version=11.4
  sync_out : Outport
  dout : Outport  Port=2
  wires:
  sync/1 -> sync_delay/1
  sync_delay/1 -> sync_out/1
  din1/1 -> addr1/1
  din2/1 -> addr1/2
  din3/1 -> dly2/1
  addr1/1 -> addr3/1
  dly2/1 -> addr3/2
  addr3/1 -> dout/1

== system s_b2a4x1kf/sys0/pkt_reord/input_control/mcnt_thresh ==
  note: we record if this is the first timestamp.
      | If it is we capture it even if out of bounds
  note: capture any new mcnts which
      | are within (1/2 buffer - 1)
      | of the previous mcnt.
      | This prevents locking onto
      | bad mcnts
  note: timeout of a bad
      | master count
      | in ~2^20 clocks
  mcnt : Inport
  en : Inport  Port=2
  AddSub : xbsIndex_r4/AddSub  mode=Addition  use_carryin=off  use_carryout=off  en=off  latency=2  precision=User Defined  arith_type=Unsigned  n_bits=n_bits_timestamp + (chan_bits-xeng_bits)  bin_pt=0  quantization=Truncate  overflow=Wrap  use_behavioral_HDL=on  hw_selection=Fabric  pipelined=off  dbl_ovrd=off  block_type=addsub
  Constant1 : xbsIndex_r4/Constant  const=(2^(window_bits - 2)) + 1  gui_display_data_type=Fixed-point  arith_type=Unsigned  n_bits=window_bits  bin_pt=0  preci_type=Single  exp_width=8  frac_width=24  explicit_period=on  period=1  equ=P=C  opselect=C  inp2=PCIN>>17  opr=+  inp1=P  carry=CIN  dbl_ovrd=off  block_type=constant
  Counter : xbsIndex_r4/Counter  cnt_type=Free Running  cnt_to=Inf  operation=Up  start_count=0  cnt_by_val=1  arith_type=Unsigned  n_bits=21  bin_pt=0  load_pin=off  rst=on  en=off  explicit_period=on  period=1  use_behavioral_HDL=off  implementation=Fabric  use_rpm=on  dbl_ovrd=off  block_type=counter
      settings: xl_area=[0, 0, 0, 0, 0, 0, 0]
  Delay : xbsIndex_r4/Delay  rst=off  infoeditControl=Selection of Reset will increase slice count due to use of real FFs and instead of SRLs  en=off  latency=2  reg_retiming=on  dbl_ovrd=off  block_type=delay
      settings: xl_area=[0, 0, 0, 0, 0, 0, 0]
  Delay1 : xbsIndex_r4/Delay  rst=off  infoeditControl=Selection of Reset will increase slice count due to use of real FFs and instead of SRLs  en=off  latency=1  reg_retiming=on  dbl_ovrd=off  block_type=delay
      settings: xl_area=[0, 0, 0, 0, 0, 0, 0]
  Gateway Out{,1..6} (7 alike) : xbsIndex_r4/Gateway Out  inherit_from_input=off  hdl_port=on  rows=1  columns=1  UseAsDAC=off  DACChannel='1'  interface=None  automatic_assignment=on  address_offset=hex2dec('00')  intf_name=''  intf_description=''  timing_constraint=None  locs_specified=off  LOCs={}  io_standard={}  block_type=gatewayout
  Inverter : xbsIndex_r4/Inverter  en=off  latency=0  dbl_ovrd=off  block_type=inv
  Logical : xbsIndex_r4/Logical  logical_function=AND  inputs=2  en=off  latency=0  precision=Full  arith_type=Unsigned  n_bits=8  bin_pt=2  align_bp=on  dbl_ovrd=off  block_type=logical
      settings: xl_area=[0, 0, 0, 0, 0, 0, 0]
  Logical1 : xbsIndex_r4/Logical  logical_function=OR  inputs=3  en=off  latency=0  precision=Full  arith_type=Unsigned  n_bits=8  bin_pt=2  align_bp=on  dbl_ovrd=off  block_type=logical
      settings: xl_area=[0, 0, 0, 0, 0, 0, 0]
  Register : xbsIndex_r4/Delay  rst=off  infoeditControl=Selection of Reset will increase slice count due to use of real FFs and instead of SRLs  en=on  latency=1  reg_retiming=on  dbl_ovrd=off  block_type=delay
  Relational : xbsIndex_r4/Relational  mode=a>b  op_type=Bool  en=off  latency=1  dbl_ovrd=off  block_type=relational
      settings: xl_area=[0, 0, 0, 0, 0, 0, 0]  block_version=10.1.3
  Relational1 : xbsIndex_r4/Relational  mode=a<=b  op_type=Bool  en=off  latency=1  dbl_ovrd=off  block_type=relational
      settings: xl_area=[0, 0, 0, 0, 0, 0, 0]  block_version=10.1.3
  Scope1 : Scope  NumInputPorts=7
  Slice : xbsIndex_r4/Slice  nbits=1  boolean_output=on  mode=Upper Bit Location + Width  bit1=0  base1=MSB of Input  bit0=0  base0=LSB of Input  dbl_ovrd=off  block_type=slice
      settings: infoedit="Extracts a given range of bits from each input sample and presents it at the output.  The output type is ordinarily unsigned with binary point at zero, but can be Boolean when the slice is one bit wide.<P><P>Hardware notes: In hardware this block costs nothing."  block_version=10.1.3
  edge_detect : Subsystem  mask(edge_detect){edge=Rising, polarity=Active High, x_in=[0 0.08 0.08 0.16 0.16 0.24 0.24 0.32 0.32 0.4], y_in=[-1 -1  1  1  1  1  1  1  1  1], x_out=[0.6 0.68 0.68 0.76 0.76 0.84 0.84 0.92 0.92 1], y_out=[-1 -1  1  1 -1 -1 -1 -1 -1 -1]}
      mask prompts: edge "Edge Type"; polarity "Output Polarity"; x_in "Input X Positions"; y_in "Input Y Positions"; x_out "Output X Positions"; y_out "Output Y Positions"
      mask help: Output is active for one-cycle after each edge of the specified type (i.e. rising, falling or both).
      mask init: same as s_b2a4x1kf/edge_detect
      settings: AttributesFormatString=|
      | rising edges
      | active high
      mask Help: Output is active for one-cycle after each edge of the specified type (i.e. rising, falling, or both).  Latency is zero.
      mask TypeOptions edge: Rising | Falling | Both
      mask TypeOptions polarity: Active High | Active Low
      mask Display:
      | plot(x_in_num,0.5+y_in_num*0.2);
      | plot(x_out_num,0.5+y_out_num*0.2);
  not_first : xbsIndex_r4/Delay  rst=off  infoeditControl=Selection of Reset will increase slice count due to use of real FFs and instead of SRLs  en=on  latency=1  reg_retiming=on  dbl_ovrd=off  block_type=delay
  maxcnt : Outport
  mcnt_timeout : Outport  Port=2
  wires:
  Relational1/1 -> Logical/2
  mcnt/1 -> Relational1/1, Relational/1, Gateway Out/1, Delay1/1
  Slice/1 -> edge_detect/1(in), Logical1/1
  Logical1/1 -> Counter/1, Register/2, Gateway Out4/1
  Logical/1 -> Logical1/2, Gateway Out2/1
  Counter/1 -> Gateway Out1/1, Slice/1
  Relational/1 -> Logical/1
  Register/1 -> AddSub/1, maxcnt/1, Gateway Out5/1, Delay/1
  AddSub/1 -> Gateway Out6/1, Relational1/2
  en/1 -> not_first/1, not_first/2
  Inverter/1 -> Gateway Out3/1, Logical1/3
  Delay1/1 -> Register/1
  Gateway Out/1 -> Scope1/1
  Gateway Out1/1 -> Scope1/2
  Gateway Out2/1 -> Scope1/3
  Gateway Out3/1 -> Scope1/4
  Gateway Out4/1 -> Scope1/5
  Gateway Out5/1 -> Scope1/6
  Gateway Out6/1 -> Scope1/7
  Delay/1 -> Relational/2
  not_first/1 -> Inverter/1
  Constant1/1 -> AddSub/2
  edge_detect/1(out) -> mcnt_timeout/1

== system s_b2a4x1kf/sys0/pkt_reord/input_control/snap ==
  in_wr_addr : Inport
  in_wr_en : Inport  Port=2
  in_max_mcnt : Inport  Port=3
  in_disc_err : Inport  Port=4
  in_timestamp : Inport  Port=5
  in_timeout_err : Inport  Port=6
  we : Inport  Port=7
  trig : Inport  Port=8
  stop : Inport  Port=9
  assert_disc_err : xbsIndex_r4/Assert  assert_type=on  type_source=Explicitly  gui_display_data_type=Boolean  arith_type=Boolean  n_bits=1  bin_pt=0  preci_type=Single  exp_width=8  frac_width=24  assert_rate=off  rate_source=Explicitly  period=1  output_port=on  block_type=assert
  assert_max_mcnt : xbsIndex_r4/Assert  assert_type=on  type_source=Explicitly  gui_display_data_type=Fixed-point  arith_type=Unsigned  n_bits=36  bin_pt=0  preci_type=Single  exp_width=8  frac_width=24  assert_rate=off  rate_source=Explicitly  period=1  output_port=on  block_type=assert
  assert_timeout_err : xbsIndex_r4/Assert  assert_type=on  type_source=Explicitly  gui_display_data_type=Boolean  arith_type=Boolean  n_bits=1  bin_pt=0  preci_type=Single  exp_width=8  frac_width=24  assert_rate=off  rate_source=Explicitly  period=1  output_port=on  block_type=assert
  assert_timestamp : xbsIndex_r4/Assert  assert_type=on  type_source=Explicitly  gui_display_data_type=Fixed-point  arith_type=Unsigned  n_bits=36  bin_pt=0  preci_type=Single  exp_width=8  frac_width=24  assert_rate=off  rate_source=Explicitly  period=1  output_port=on  block_type=assert
  assert_wr_addr : xbsIndex_r4/Assert  assert_type=on  type_source=Explicitly  gui_display_data_type=Fixed-point  arith_type=Unsigned  n_bits=8  bin_pt=0  preci_type=Single  exp_width=8  frac_width=24  assert_rate=off  rate_source=Explicitly  period=1  output_port=on  block_type=assert
  assert_wr_en : xbsIndex_r4/Assert  assert_type=on  type_source=Explicitly  gui_display_data_type=Boolean  arith_type=Boolean  n_bits=1  bin_pt=0  preci_type=Single  exp_width=8  frac_width=24  assert_rate=off  rate_source=Explicitly  period=1  output_port=on  block_type=assert
  buscreate : Subsystem  AncestorBlock=casper_library_flow_control/bus_create  mask(bus_create){inputNum=6}
      mask prompts: inputNum "Number of inputs:"
      mask init:
      | bus_create_init(gcb,...
      |     'inputNum', inputNum);
  ss : Subsystem  Tag=casper:snapshot  AncestorBlock=casper_library_scopes/snapshot  mask(snapshot){storage=bram, dram_dimm=2, dram_clock=250, nsamples=13, data_width=128, offset=off, circap=on, value=off, ext_arm=off, ext_circ=off, provide_outputs=off, use_dsp48=on}
      mask prompts: storage "Storage medium"; dram_dimm "DRAM dimm"; dram_clock "DRAM clock rate"; nsamples "Number of Samples (2^?)"; data_width "Data width"; offset "Start delay support"; circap "Circular capture support"; value "Extra value capture support"; ext_arm "External arm support"; ext_circ "External circular capture support"; provide_outputs "Provide outputs"; use_dsp48 "Use DSP48s to implement counters"
      mask help:
      | Standard snap block, but with the following optional extras;
      |  1) Optionally delay the fabric trigger by a user-specified number of valids.
      |  2) Capture continuously after a trigger until a stop pulse is received. Data is captured into BRAM continuously, with old data being overwritten until a stop command is received. Then stop capturing when memory is filled. This enables you to get some data before and some data after the stop pulse. Use the 'tr_en_cnt' register to determine where you are in your vector. 'Addr' register's MSb now indicates 'busy capturing'.
      |  3) Optionally capture a value on an input port to a register at the same time as the first data sample.
      |  4) Implement counters using DSP48Es to save resources.
      mask init: same as s_b2a4x1kf/snap_gbe0_rx/ss
      settings: AttributesFormatString=|
      | 128 wide, 8192 deep
      | debugID: 14195851
      mask TypeOptions storage: bram | dram
      mask Callback storage: snapshot_callback();
      mask TypeOptions dram_dimm: 1 | 2 | 3 | 4
      mask TypeOptions dram_clock: 200 | 250 | 266 | 300 | 333
      mask TypeOptions data_width: 8 | 16 | 32 | 64 | 128
  arm_out : Outport
  wires:
  ss/1(arm_out) -> arm_out/1
  buscreate/1(bus_out) -> ss/1(din)
  in_wr_addr/1 -> assert_wr_addr/1
  assert_wr_addr/1 -> buscreate/1(in1)
  in_wr_en/1 -> assert_wr_en/1
  assert_wr_en/1 -> buscreate/2(in2)
  in_max_mcnt/1 -> assert_max_mcnt/1
  assert_max_mcnt/1 -> buscreate/3(in3)
  in_disc_err/1 -> assert_disc_err/1
  assert_disc_err/1 -> buscreate/4(in4)
  in_timestamp/1 -> assert_timestamp/1
  assert_timestamp/1 -> buscreate/5(in5)
  in_timeout_err/1 -> assert_timeout_err/1
  assert_timeout_err/1 -> buscreate/6(in6)
  we/1 -> ss/2(we)
  trig/1 -> ss/3(trig)
  stop/1 -> ss/4(stop)
